simulink model "ADCS_Software_test"  (R2025b)
settings: Solver=VariableStepAuto  StartTime=0.0  StopTime=t0*1.5  FixedStep=0.1  MaxStep=0.1  RelTol=1e-3
values from neighbouring files (symbols this model uses):
  B = [1 0 0]    [parameters.m]
  h0 = [1 1 1]*0.5    [parameters.m]
  h_max = 1.47    [parameters.m]
  I_RW = 1    [parameters.m]
  k_desat = 1    [parameters.m]
  kd_detumble = 1    [parameters.m]
  kd_hold = 1    [parameters.m]
  kd_point = 20    [parameters.m]
  kd_slew_fast = 1    [parameters.m]
  kd_slew_slow = 1    [parameters.m]
  kd_spin = 0    [parameters.m]
  kp_hold = 1    [parameters.m]
  kp_point = 2    [parameters.m]
  kp_slew_fast = 1    [parameters.m]
  kp_slew_slow = 1    [parameters.m]
  kp_spin = 1    [parameters.m]
  omega_0 = [0 0 0.0011]    [parameters.m]
  omega_thr = 0.1    [parameters.m]    (also in run_ADCS_FSM_test_suite.m = 1)
  omega_zero = 0.001    [parameters.m]
  P = satellite_params()    [individual_test_with_dynamics.m]    (also in parameters.m; test.m = thrusters(:, 1:3))
  q0 = [sqrt(0.5) -sqrt(0.5) 0 0]    [parameters.m]
  ts = 0.1    [parameters.m]
undefined symbols (not defined in the file or in its folder): IAU
libraries: matrix_library x10, simulink x3, sim3dlib x2, aerolibutil x2, aerolibtransform2 x1
(part 2 of 2)

== stateflow chart ADCS_Software_test/Subsystem3/Mode manager/Mode Manager/ACS_Manager ==
  state ACS_DETUMBLE
    entry:
    actual_acs = uint8(1);
  state ACS_POINT
    entry:
    actual_acs = uint8(2);
  state ACS_IDLE
    entry:
    actual_acs = uint8(0);
  state ACS_SLEW_SLOW
    entry:
    actual_acs = uint8(4);
  state ACS_DESAT
    entry:
    actual_acs = uint8(7);
    %exit:
    %desaturated = 1;
  state ACS_HOLD
    entry:
    actual_acs = uint8(3);
  state ACS_OPTICAL
    entry:
    actual_acs = uint8(8);
  state ACS_SPIN
    entry:
    actual_acs = uint8(6);
  state ACS_SLEW_FAST
    entry:
    actual_acs = uint8(5);
  state ACS_SAFE
    entry:
    actual_acs = uint8(9);
  ACS_SLEW_SLOW -> ACS_DESAT [order 3] : [wheels_saturated && ~energy_low]
  ACS_OPTICAL -> ACS_POINT [order 3] : [~optical_target_available &&...
      |  ~energy_low]
  (junction 25) -> ACS_DETUMBLE [order 2] : [desired_acs == uint8(1) ...
      | ||~detumbled]
  ACS_DETUMBLE -> (junction 25) : [desired_acs ~= uint8(1) && zero_omega]
  ACS_POINT -> ACS_SAFE [order 2] : [energy_low || ~reference_available ||...
      |  actual_ephem == uint8(0)]%~detumbled ||
  ACS_POINT -> (junction 25) [order 1] : [desired_acs ~= uint8(2) ||...
      | ~detumbled]
  (junction 25) -> ACS_POINT [order 3] : [desired_acs == uint8(2) && detumbled && desaturated]
  (junction 25) -> ACS_IDLE [order 1] : [desired_acs == uint8(0)]
  (default) -> ACS_IDLE
  ACS_IDLE -> (junction 25) : [desired_acs ~= uint8(0)]
  (junction 25) -> ACS_SLEW_SLOW [order 5] : [desired_acs == uint8(4)]
  ACS_SLEW_SLOW -> (junction 25) [order 1] : [desired_acs ~= uint8(4)]
  ACS_SLEW_SLOW -> ACS_SAFE [order 2] : [energy_low || ~detumbled ||...
      |  actual_ephem == uint8(0)]
  ACS_HOLD -> (junction 25) [order 1] : [desired_acs ~= uint8(3)]
  ACS_DESAT -> (junction 25) [order 1] : [desired_acs ~= uint8(7) &&...
      |  desaturated && recovery_ready &&...
      |  ~energy_low]
  (junction 25) -> ACS_HOLD [order 4] : [desired_acs == uint8(3)]
  (junction 25) -> ACS_DESAT [order 8] : [desired_acs == uint8(7)||wheels_saturated]
  ACS_OPTICAL -> (junction 25) [order 1] : [desired_acs ~= uint8(8) && optical_target_available]
  (junction 25) -> ACS_OPTICAL [order 9] : [desired_acs == uint8(8)]
  (junction 25) -> ACS_SLEW_FAST [order 6] : [desired_acs == uint8(5)]
  ACS_SLEW_FAST -> (junction 25) [order 1] : [desired_acs ~= uint8(5)]
  ACS_SAFE -> (junction 25) : [desired_acs ~= uint8(9) &&...
      |  ~energy_low && recovery_ready &&...
      |  sun_sensor_valid && ~((desired_acs == uint8(2)) &&...
      |  ~reference_available) && ~((desired_acs == uint8(6)) &&...
      |  (~spin_feasible || ~spin_axis_available))]
  (junction 25) -> ACS_SAFE [order 10] : [desired_acs == uint8(9)]
  (junction 25) -> ACS_SPIN [order 7] : [desired_acs == uint8(6)]
  ACS_SPIN -> (junction 25) [order 2] : [desired_acs ~= uint8(6)]
  ACS_DESAT -> ACS_SAFE [order 2] : [energy_low]
  ACS_SLEW_FAST -> ACS_DESAT [order 3] : [wheels_saturated && ~energy_low]
  ACS_HOLD -> ACS_SAFE [order 2] : [energy_low ||...
      |  ~detumbled ||...
      |  actual_ephem == uint8(0)]
  ACS_OPTICAL -> ACS_SAFE [order 2] : [energy_low]
  ACS_SPIN -> ACS_SAFE [order 1] : [energy_low || ~spin_feasible ||...
      |  ~spin_axis_available]
  ACS_SLEW_FAST -> ACS_SAFE [order 2] : [energy_low || ~detumbled ||...
      |  actual_ephem == uint8(0)]
  data: desired_acs input uint8; actual_ephem input uint8; detumbled input boolean; zero_omega input; reference_available input boolean; energy_low input boolean; recovery_ready input boolean; wheels_saturated input boolean; desaturated input boolean; spin_feasible input boolean; spin_axis_available input boolean; optical_target_available input boolean; sun_sensor_valid input boolean; actual_acs output uint8 =0

== stateflow chart ADCS_Software_test/Subsystem3/Mode manager/Status_Manager ==
  state STATUS
    during:
    mode_degraded = (actual_ephem ~= desired_ephem) || (actual_ads ~= desired_ads) || (actual_frame ~= desired_frame) || (actual_acs ~= desired_acs);
  (default) -> STATUS
  data: desired_ephem input uint8; desired_ads input uint8; desired_frame input uint8; desired_acs input uint8; actual_ephem input uint8; actual_ads input uint8; actual_frame input uint8; actual_acs input uint8; mode_degraded output boolean =0

== stateflow chart ADCS_Software_test/Subsystem3/Mode manager/Mode Manager/Ephemeris_Manager ==
  state EPHEM_IDLE
    entry:
    actual_ephem = uint8(0);
  state EPHEM_GPS
    entry:
    actual_ephem = uint8(2);
  state EPHEM_TLE
    entry:
    actual_ephem = uint8(1);
  EPHEM_GPS -> EPHEM_IDLE [order 1] : [desired_ephem == uint8(0)]
  EPHEM_IDLE -> EPHEM_GPS [order 2] : [desired_ephem == uint8(2)...
      |  && gps_valid]
  (default) -> EPHEM_IDLE
  EPHEM_IDLE -> EPHEM_TLE [order 1] : [desired_ephem == uint8(1) ||...
      |  (desired_ephem == uint8(2) &&...
      |  ~gps_valid && ~tle_error_high)]
  EPHEM_TLE -> EPHEM_IDLE [order 1] : [desired_ephem == uint8(0)...
      |  || tle_error_high]
  EPHEM_GPS -> EPHEM_TLE [order 2] : [desired_ephem == uint8(1) ||...
      |  ~gps_valid]
  EPHEM_TLE -> EPHEM_GPS [order 2] : [desired_ephem == uint8(2) && gps_valid]
  data: desired_ephem input uint8; gps_valid input boolean; tle_error_high input boolean; actual_ephem output uint8 =0

== stateflow chart ADCS_Software_test/Subsystem3/Mode manager/Mode Manager/ADS_Manager ==
  state ADS_IDLE
    entry:
    actual_ads = uint8(0);
  state ADS_UKF_FINE
    entry:
    actual_ads = uint8(2);
  state ADS_UKF_COARSE
    entry:
    actual_ads = uint8(1);
  ADS_UKF_FINE -> ADS_IDLE [order 2] : [desired_ads == uint8(0) || ads_fault]
  ADS_IDLE -> ADS_UKF_FINE [order 2] : [desired_ads == uint8(2) &&...
      |  ads_fine_allowed && ~ads_fault]
  (default) -> ADS_IDLE
  ADS_UKF_COARSE -> ADS_IDLE [order 1] : [desired_ads == uint8(0) || ads_fault]
  ADS_IDLE -> ADS_UKF_COARSE [order 1] : [desired_ads == uint8(1) ||...
      |  (desired_ads == uint8(2) &&...
      |  ~ads_fine_allowed)]
  ADS_UKF_FINE -> ADS_UKF_COARSE [order 1] : [desired_ads == uint8(1) ||...
      |  ~ads_fine_allowed]
  ADS_UKF_COARSE -> ADS_UKF_FINE [order 2] : [desired_ads == uint8(2) &&...
      |  ads_fine_allowed && ~ads_fault]
  data: desired_ads input uint8; ads_fine_allowed input boolean; ads_fault input boolean; actual_ads output uint8 =0

== stateflow chart ADCS_Software_test/Subsystem3/Mode manager/Mode Manager/Mission_Mode_Manager ==
  state M_DETUMBLE
    entry:
    desired_ephem = uint8(0);
    desired_ads = uint8(1);
    desired_frame = uint8(0);
    desired_acs = uint8(1);
    %desired_actuator = uint8(3);
  state M_SAFE_SUN
    entry:
    desired_ephem = uint8(0);
    desired_ads = uint8(0);
    desired_frame = uint8(0);
    desired_acs = uint8(9);
    %desired_actuator = uint8(2);
  state M_Y_SPIN
    entry:
    desired_ephem = uint8(2);
    desired_ads = uint8(1);
    desired_frame = uint8(1);
    desired_acs = uint8(6);
    %desired_actuator = uint8(2);
  state M_IDLE
    entry:
    desired_ephem = uint8(0);
    desired_ads = uint8(0);
    desired_frame = uint8(0);
    desired_acs = uint8(0);
    %desired_actuator = uint8(0);
  state M_MINMAX_DRAG
    entry:
    desired_ephem = uint8(2);
    desired_ads = uint8(2);
    desired_frame = uint8(3);
    %desired_frame = uint8(3 + 2 * drag_use_vnb);
    desired_acs = uint8(2);
    %desired_actuator = uint8(2);
  state M_POINT_NADIR
    entry:
    desired_ephem = uint8(2);
    desired_ads = uint8(2);
    desired_frame = uint8(3);
    desired_acs = uint8(2);
    %desired_actuator = uint8(2);
  state M_SLEW_FIXED
    entry:
    desired_ephem = uint8(2);
    desired_ads = uint8(2);
    desired_frame = uint8(2);
    desired_acs = uint8(4);
    %desired_actuator = uint8(2);
  state M_SLEW_FASTEST
    entry:
    desired_ephem = uint8(2);
    desired_ads = uint8(2);
    desired_frame = uint8(2);
    desired_acs = uint8(5);
    %desired_actuator = uint8(3);
  state M_POINT_EARTH_TARGET
    entry:
    desired_ephem = uint8(2);
    desired_ads = uint8(2);
    desired_frame = uint8(4);
    desired_acs = uint8(2);
    %desired_actuator = uint8(2);
  state M_TDI
    entry:
    desired_ephem = uint8(2);
    desired_ads = uint8(2);
    desired_frame = uint8(6);
    desired_acs = uint8(2);
    %desired_actuator = uint8(2);
  state M_POINT_SUN
    entry:
    desired_ephem = uint8(2);
    desired_ads = uint8(2);
    desired_frame = uint8(2);
    desired_acs = uint8(2);
    %desired_actuator = uint8(2);
  state M_INTERSAT_TRACK
    entry:
    desired_ephem = uint8(2);
    desired_ads = uint8(2);
    desired_frame = uint8(2);
    desired_acs = uint8(2 + 6 * intersat_sensor_tracking);
    %desired_actuator = uint8(2);
  M_DETUMBLE -> (junction 28) : [mission_cmd ~= uint8(1)]
  (junction 28) -> M_DETUMBLE [order 2] : [mission_cmd == uint8(1)]
  M_Y_SPIN -> (junction 28) : [mission_cmd ~= uint8(3)]
  M_SAFE_SUN -> (junction 28) : [mission_cmd ~= uint8(2)]
  (junction 28) -> M_SAFE_SUN [order 3] : [mission_cmd == uint8(2)]
  M_IDLE -> (junction 28) : [mission_cmd ~= uint8(0)]
  (default) -> M_IDLE
  (junction 28) -> M_IDLE [order 1] : [mission_cmd == uint8(0)]
  (junction 28) -> M_Y_SPIN [order 4] : [mission_cmd == uint8(3)]
  (junction 28) -> M_MINMAX_DRAG [order 12] : [mission_cmd == uint8(11)]
  M_MINMAX_DRAG -> (junction 28) : [mission_cmd ~= uint8(11)]
  (junction 28) -> M_POINT_NADIR [order 5] : [mission_cmd == uint8(4)]
  M_POINT_NADIR -> (junction 28) : [mission_cmd ~= uint8(4)]
  (junction 28) -> M_SLEW_FIXED [order 8] : [mission_cmd == uint8(7)]
  M_SLEW_FASTEST -> (junction 28) : [mission_cmd ~= uint8(8)]
  (junction 28) -> M_SLEW_FASTEST [order 9] : [mission_cmd == uint8(8)]
  M_SLEW_FIXED -> (junction 28) : [mission_cmd ~= uint8(7)]
  (junction 28) -> M_POINT_EARTH_TARGET [order 7] : [mission_cmd == uint8(6)]
  (junction 28) -> M_POINT_SUN [order 6] : [mission_cmd == uint8(5)]
  M_POINT_EARTH_TARGET -> (junction 28) : [mission_cmd ~= uint8(6)]
  M_POINT_SUN -> (junction 28) : [mission_cmd ~= uint8(5)]
  (junction 28) -> M_INTERSAT_TRACK [order 10] : [mission_cmd == uint8(9)]
  (junction 28) -> M_TDI [order 11] : [mission_cmd == uint8(10)]
  M_INTERSAT_TRACK -> (junction 28) : [mission_cmd ~= uint8(9)]
  M_TDI -> (junction 28) : [mission_cmd ~= uint8(10)]
  data: mission_cmd input uint8; intersat_sensor_tracking input boolean; desired_ephem output uint8 =0; desired_ads output uint8 =0; desired_frame output uint8 =0; desired_acs output uint8 =0
